simulink model "acf_sea_pad_research_20261006"  (R2026b)
settings: Solver=ode4  StopTime=p.stopTime  FixedStep=2.5000000000000002e-06
model workspace (MAT data in the model file):
  p : object (value not decoded)
  replayInputs = [0 0.0001 0.0002 0.0003 0.0004 0.0005 0.0006 0.0007 0.0008 0.0009 0.001 0.0011 ... (60003 elements, 20001x3)]
symbols that are objects in the model workspace (value not decoded): p
libraries: simulink x1
(part 2 of 2)

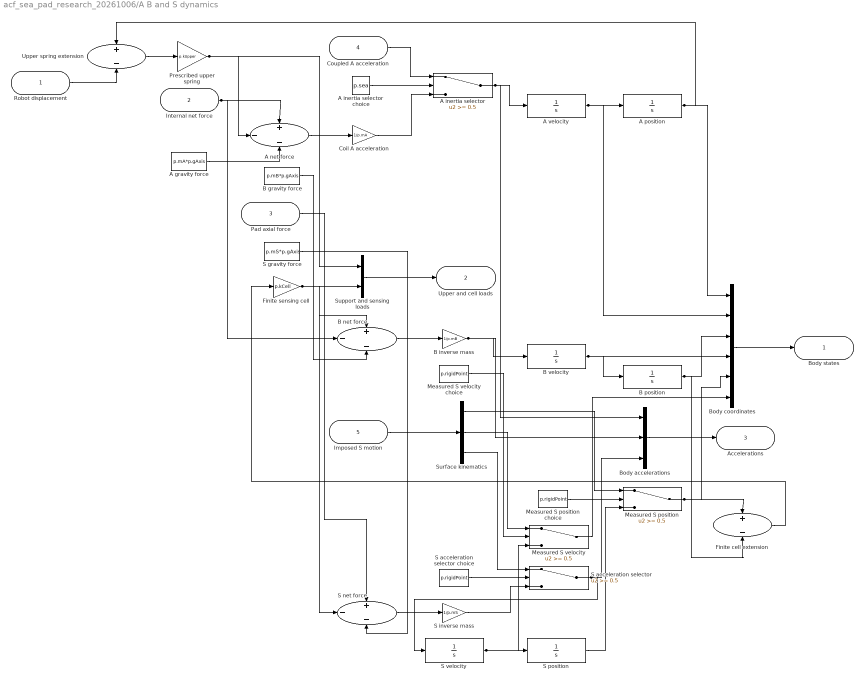
== system acf_sea_pad_research_20261006/A B and S dynamics ==
  Robot displacement : Inport
  Internal net force : Inport  Port=2
  Pad axial force : Inport  Port=3
  Coupled A acceleration : Inport  Port=4
  Imposed S motion : Inport  Port=5
  A gravity force : Constant  Value=p.mA*p.gAxis
  A inertia selector : Switch  Threshold=0.5  SaturateOnIntegerOverflow=off  InputSameDT=off
  A inertia selector choice : Constant  Value=p.sea
  A net force : Sum  Inputs=+--
  A position : Integrator  InitialCondition=p.initial(1)
  A velocity : Integrator  InitialCondition=p.initial(2)
  B gravity force : Constant  Value=p.mB*p.gAxis
  B inverse mass : Gain  Gain=1/p.mB
  B net force : Sum  Inputs=+--
  B position : Integrator  InitialCondition=p.initial(3)
  B velocity : Integrator  InitialCondition=p.initial(4)
  Body accelerations : Mux  Inputs=3
  Body coordinates : Mux  Inputs=6
  Coil A acceleration : Gain  Gain=1/p.mA
  Finite cell extension : Sum  Inputs=+-
  Finite sensing cell : Gain  Gain=p.kCell
  Measured S position : Switch  Threshold=0.5  SaturateOnIntegerOverflow=off  InputSameDT=off
  Measured S position choice : Constant  Value=p.rigidPoint
  Measured S velocity : Switch  Threshold=0.5  SaturateOnIntegerOverflow=off  InputSameDT=off
  Measured S velocity choice : Constant  Value=p.rigidPoint
  Prescribed upper spring : Gain  Gain=p.kUpper
  S acceleration selector : Switch  Threshold=0.5  SaturateOnIntegerOverflow=off  InputSameDT=off
  S acceleration selector choice : Constant  Value=p.rigidPoint
  S gravity force : Constant  Value=p.mS*p.gAxis
  S inverse mass : Gain  Gain=1/p.mS
  S net force : Sum  Inputs=+--
  S position : Integrator  InitialCondition=p.initial(5)
  S velocity : Integrator  InitialCondition=p.initial(6)
  Support and sensing loads : Mux  Inputs=2
  Surface kinematics : Demux  Outputs=3
  Upper spring extension : Sum  Inputs=+-
  Body states : Outport
  Upper and cell loads : Outport  Port=2
  Accelerations : Outport  Port=3
  wires:
  Finite cell extension/1 -> Finite sensing cell/1
  Body accelerations/1 -> Accelerations/1
  B position/1 -> Body coordinates/3, Finite cell extension/2
  A position/1 -> Body coordinates/1, Upper spring extension/1
  S position/1 -> Measured S position/3
  Coil A acceleration/1 -> A inertia selector/3
  Finite sensing cell/1 -> Support and sensing loads/2, S net force/2, B net force/1
  Measured S velocity/1 -> Body coordinates/6
  A net force/1 -> Coil A acceleration/1
  A inertia selector/1 -> A velocity/1, Body accelerations/1
  Measured S position/1 -> Body coordinates/5, Finite cell extension/1
  A inertia selector choice/1 -> A inertia selector/2
  A gravity force/1 -> A net force/3
  S acceleration selector choice/1 -> S acceleration selector/2
  Support and sensing loads/1 -> Upper and cell loads/1
  Imposed S motion/1 -> Surface kinematics/1
  Measured S velocity choice/1 -> Measured S velocity/2
  Pad axial force/1 -> S net force/1
  Surface kinematics/2 -> Measured S velocity/1
  Coupled A acceleration/1 -> A inertia selector/1
  Prescribed upper spring/1 -> A net force/2, Support and sensing loads/1
  S velocity/1 -> Measured S velocity/3, S position/1
  Upper spring extension/1 -> Prescribed upper spring/1
  Robot displacement/1 -> Upper spring extension/2
  Surface kinematics/3 -> S acceleration selector/1
  Body coordinates/1 -> Body states/1
  S gravity force/1 -> S net force/3
  B net force/1 -> B inverse mass/1
  S inverse mass/1 -> S acceleration selector/3
  S net force/1 -> S inverse mass/1
  Internal net force/1 -> B net force/2, A net force/1
  B inverse mass/1 -> B velocity/1, Body accelerations/2
  Surface kinematics/1 -> Measured S position/1
  B gravity force/1 -> B net force/3
  A velocity/1 -> A position/1, Body coordinates/2
  B velocity/1 -> B position/1, Body coordinates/4
  S acceleration selector/1 -> Body accelerations/3, S velocity/1
  Measured S position choice/1 -> Measured S position/2

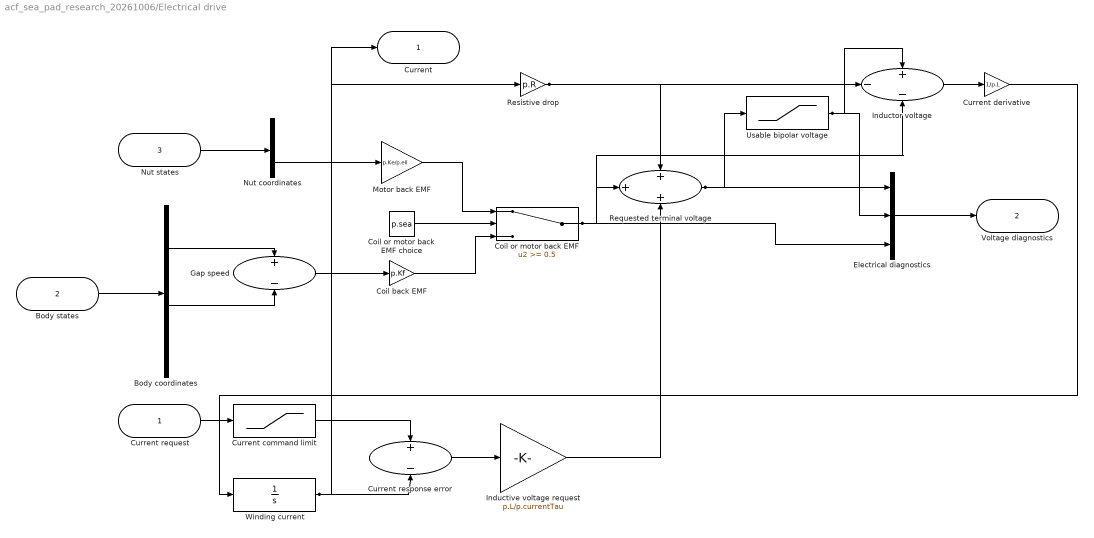
== system acf_sea_pad_research_20261006/Electrical drive ==
  Current request : Inport
  Body states : Inport  Port=2
  Nut states : Inport  Port=3
  Body coordinates : Demux  Outputs=6
  Coil back EMF : Gain  Gain=p.Kf
  Coil or motor back EMF : Switch  Threshold=0.5  SaturateOnIntegerOverflow=off  InputSameDT=off
  Coil or motor back EMF choice : Constant  Value=p.sea
  Current command limit : Saturate  UpperLimit=p.Imax  LowerLimit=-p.Imax
  Current derivative : Gain  Gain=1/p.L
  Current response error : Sum  Inputs=+-
  Electrical diagnostics : Mux  Inputs=3
  Gap speed : Sum  Inputs=+-
  Inductive voltage request : Gain  Gain=p.L/p.currentTau
  Inductor voltage : Sum  Inputs=+--
  Motor back EMF : Gain  Gain=p.Ke/p.ell
  Nut coordinates : Demux  Outputs=2
  Requested terminal voltage : Sum  Inputs=+++
  Resistive drop : Gain  Gain=p.R
  Usable bipolar voltage : Saturate  UpperLimit=p.Vmax  LowerLimit=-p.Vmax
  Winding current : Integrator  InitialCondition=p.initial(9)
  Current : Outport
  Voltage diagnostics : Outport  Port=2
  wires:
  Current derivative/1 -> Winding current/1
  Electrical diagnostics/1 -> Voltage diagnostics/1
  Inductor voltage/1 -> Current derivative/1
  Inductive voltage request/1 -> Requested terminal voltage/3
  Resistive drop/1 -> Requested terminal voltage/1, Inductor voltage/2
  Body states/1 -> Body coordinates/1
  Usable bipolar voltage/1 -> Electrical diagnostics/2, Inductor voltage/1
  Nut states/1 -> Nut coordinates/1
  Body coordinates/2 -> Gap speed/1
  Coil or motor back EMF/1 -> Requested terminal voltage/2, Inductor voltage/3, Electrical diagnostics/3
  Body coordinates/4 -> Gap speed/2
  Current request/1 -> Current command limit/1
  Current command limit/1 -> Current response error/1
  Nut coordinates/2 -> Motor back EMF/1
  Current response error/1 -> Inductive voltage request/1
  Gap speed/1 -> Coil back EMF/1
  Winding current/1 -> Current/1, Current response error/2, Resistive drop/1
  Coil or motor back EMF choice/1 -> Coil or motor back EMF/2
  Motor back EMF/1 -> Coil or motor back EMF/1
  Requested terminal voltage/1 -> Usable bipolar voltage/1, Electrical diagnostics/1
  Coil back EMF/1 -> Coil or motor back EMF/3

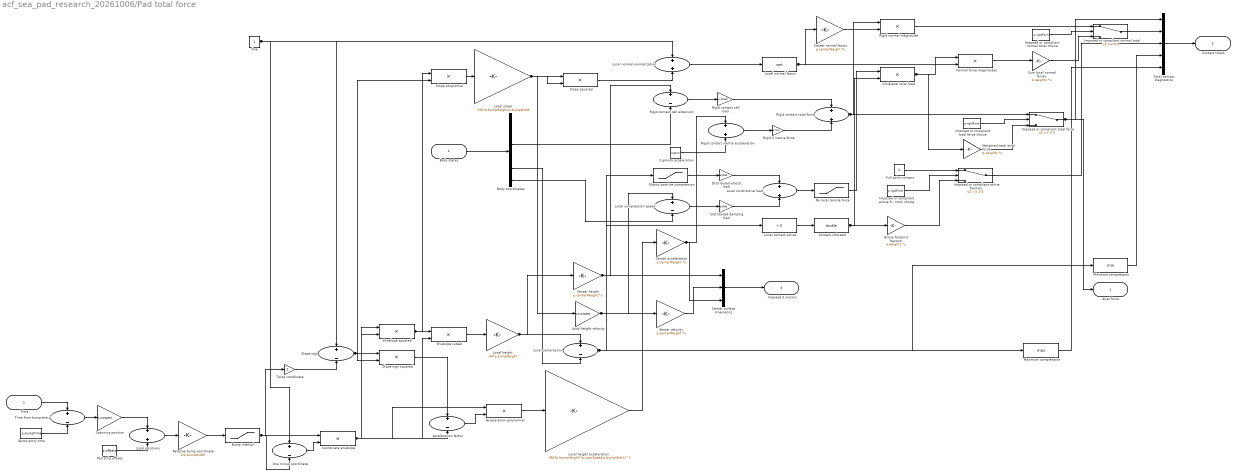
== system acf_sea_pad_research_20261006/Pad total force ==
  Time : Inport
  Body states : Inport  Port=2
  Acceleration factor : Sum  Inputs=+-
  Acceleration polynomial : Product  Inputs=**
  Active footprint fraction : Gain  Gain=p.weights  Multiplication=Matrix(K*u)
  Body coordinates : Demux  Outputs=6
  Bump entry time : Constant  Value=p.bumpTime
  Bump interval : Saturate  UpperLimit=1  LowerLimit=0
  Center acceleration : Gain  Gain=p.centerWeight  Multiplication=Matrix(K*u)
  Center height : Gain  Gain=p.centerWeight  Multiplication=Matrix(K*u)
  Center normal factor : Gain  Gain=p.centerWeight  Multiplication=Matrix(K*u)
  Center surface kinematics : Mux  Inputs=3
  Center velocity : Gain  Gain=p.centerWeight  Multiplication=Matrix(K*u)
  Contact indicator : DataTypeConversion  OutDataTypeStr=double  SaturateOnIntegerOverflow=off  RndMeth=Floor
  Coordinate envelope : Product  Inputs=**
  Distributed damping load : Gain  Gain=p.cPad
  Distributed elastic load : Gain  Gain=p.kPad
  Elastic positive compression : Saturate  UpperLimit=inf  LowerLimit=0
  Envelope cubed : Product  Inputs=**
  Envelope squared : Product  Inputs=**
  Full point contact : Constant
  Imposed or compliant active fraction : Switch  Threshold=0.5  SaturateOnIntegerOverflow=off  InputSameDT=off
  Imposed or compliant active fraction choice : Constant  Value=p.rigidPoint
  Imposed or compliant normal total : Switch  Threshold=0.5  SaturateOnIntegerOverflow=off  InputSameDT=off
  Imposed or compliant normal total choice : Constant  Value=p.rigidPoint
  Imposed or compliant total force : Switch  Threshold=0.5  SaturateOnIntegerOverflow=off  InputSameDT=off
  Imposed or compliant total force choice : Constant  Value=p.rigidPoint
  Local compression : Sum  Inputs=+-
  Local compression speed : Sum  Inputs=+-
  Local constitutive load : Sum
  Local contact active : simulink/Logic and Bit Operations/Compare To Constant  relop=>  const=0  OutDataTypeStr=boolean
  Local height : Gain  Gain=64*p.bumpHeight
  Local height acceleration : Gain  Gain=384*p.bumpHeight*(p.scanSpeed/p.bumpWidth)^2
  Local height velocity : Gain  Gain=p.scanSpeed
  Local normal factor : Sqrt
  Local normal normalization : Sum
  Local positions : Sum
  Local slope : Gain  Gain=192*p.bumpHeight/p.bumpWidth
  Maximum compression : MinMax  Function=max
  Minimum compression : MinMax
  No local tensile force : Saturate  UpperLimit=inf  LowerLimit=0
  Normal force magnitudes : Product  Inputs=**
  One : Constant
  One minus coordinate : Sum  Inputs=+-
  Pad strip offsets : Constant  Value=p.offsets
  Relative bump coordinate : Gain  Gain=1/p.bumpWidth
  Rigid S inertia force : Gain  Gain=p.mS
  Rigid contact cell extension : Sum  Inputs=+-
  Rigid contact cell load : Gain  Gain=p.kCell
  Rigid contact inertia acceleration : Sum
  Rigid contact total force : Sum
  Rigid normal magnitude : Product  Inputs=**
  S gravity acceleration : Constant  Value=p.gAxis
  Scanning position : Gain  Gain=p.scanSpeed
  Slope polynomial : Product  Inputs=**
  Slope sign : Sum  Inputs=+-
  Slope sign squared : Product  Inputs=**
  Slope squared : Product  Inputs=**
  Sum local normal forces : Gain  Gain=p.weights  Multiplication=Matrix(K*u)
  Time from bump entry : Sum  Inputs=+-
  Total contact diagnostics : Mux  Inputs=5
  Twice coordinate : Gain  Gain=2
  Unilateral local load : Product  Inputs=**
  Weighted total axial force : Gain  Gain=p.weights  Multiplication=Matrix(K*u)
  Axial force : Outport
  Contact totals : Outport  Port=2
  Imposed S motion : Outport  Port=3
  wires:
  Minimum compression/1 -> Total contact diagnostics/4
  Imposed or compliant normal total/1 -> Total contact diagnostics/2
  Maximum compression/1 -> Total contact diagnostics/5
  Local compression/1 -> Elastic positive compression/1, Maximum compression/1, Local contact active/1, Minimum compression/1
  Slope squared/1 -> Local normal normalization/2
  Acceleration polynomial/1 -> Local height acceleration/1
  Distributed damping load/1 -> Local constitutive load/2
  Local height/1 -> Center height/1, Local compression/1
  Elastic positive compression/1 -> Distributed elastic load/1
  Center acceleration/1 -> Center surface kinematics/3, Rigid contact inertia acceleration/1
  Center normal factor/1 -> Rigid normal magnitude/2
  Imposed or compliant active fraction choice/1 -> Imposed or compliant active fraction/2
  Slope polynomial/1 -> Local slope/1
  Local normal normalization/1 -> Local normal factor/1
  Envelope cubed/1 -> Local height/1
  Local contact active/1 -> Contact indicator/1
  Slope sign squared/1 -> Acceleration factor/1
  Normal force magnitudes/1 -> Sum local normal forces/1
  Imposed or compliant active fraction/1 -> Total contact diagnostics/3
  Sum local normal forces/1 -> Imposed or compliant normal total/3
  Time from bump entry/1 -> Scanning position/1
  Body coordinates/5 -> Local compression/2
  Body coordinates/3 -> Rigid contact cell extension/2
  Bump entry time/1 -> Time from bump entry/2
  Scanning position/1 -> Local positions/1
  Twice coordinate/1 -> Slope sign/2
  Total contact diagnostics/1 -> Contact totals/1
  Center height/1 -> Center surface kinematics/1, Rigid contact cell extension/1
  Pad strip offsets/1 -> Local positions/2
  Contact indicator/1 -> Active footprint fraction/1, Unilateral local load/2
  Local positions/1 -> Relative bump coordinate/1
  One minus coordinate/1 -> Coordinate envelope/2
  Relative bump coordinate/1 -> Bump interval/1
  Slope sign/1 -> Slope sign squared/2, Slope polynomial/2, Slope sign squared/1
  Local slope/1 -> Slope squared/2, Slope squared/1, Local height velocity/1
  Acceleration factor/1 -> Acceleration polynomial/2
  Bump interval/1 -> Twice coordinate/1, One minus coordinate/2, Coordinate envelope/1
  Time/1 -> Time from bump entry/1
  Imposed or compliant total force/1 -> Axial force/1, Total contact diagnostics/1
  Rigid contact inertia acceleration/1 -> Rigid S inertia force/1
  Coordinate envelope/1 -> Envelope squared/1, Acceleration factor/2, Envelope squared/2, Acceleration polynomial/1, Envelope cubed/2
  Envelope squared/1 -> Slope polynomial/1, Envelope cubed/1
  Body states/1 -> Body coordinates/1
  Local normal factor/1 -> Center normal factor/1, Normal force magnitudes/2
  Active footprint fraction/1 -> Imposed or compliant active fraction/3
  Local height acceleration/1 -> Center acceleration/1
  One/1 -> Slope sign/1, Local normal normalization/1, One minus coordinate/1
  Center surface kinematics/1 -> Imposed S motion/1
  S gravity acceleration/1 -> Rigid contact inertia acceleration/2
  Local constitutive load/1 -> No local tensile force/1
  Local compression speed/1 -> Distributed damping load/1
  Rigid S inertia force/1 -> Rigid contact total force/2
  Center velocity/1 -> Center surface kinematics/2
  Unilateral local load/1 -> Normal force magnitudes/1, Weighted total axial force/1
  Imposed or compliant normal total choice/1 -> Imposed or compliant normal total/2
  Body coordinates/6 -> Local compression speed/2
  Rigid contact cell load/1 -> Rigid contact total force/1
  Distributed elastic load/1 -> Local constitutive load/1
  Local height velocity/1 -> Center velocity/1, Local compression speed/1
  Rigid contact total force/1 -> Rigid normal magnitude/1, Imposed or compliant total force/1
  No local tensile force/1 -> Unilateral local load/1
  Weighted total axial force/1 -> Imposed or compliant total force/3
  Rigid normal magnitude/1 -> Imposed or compliant normal total/1
  Imposed or compliant total force choice/1 -> Imposed or compliant total force/2
  Rigid contact cell extension/1 -> Rigid contact cell load/1
  Full point contact/1 -> Imposed or compliant active fraction/1

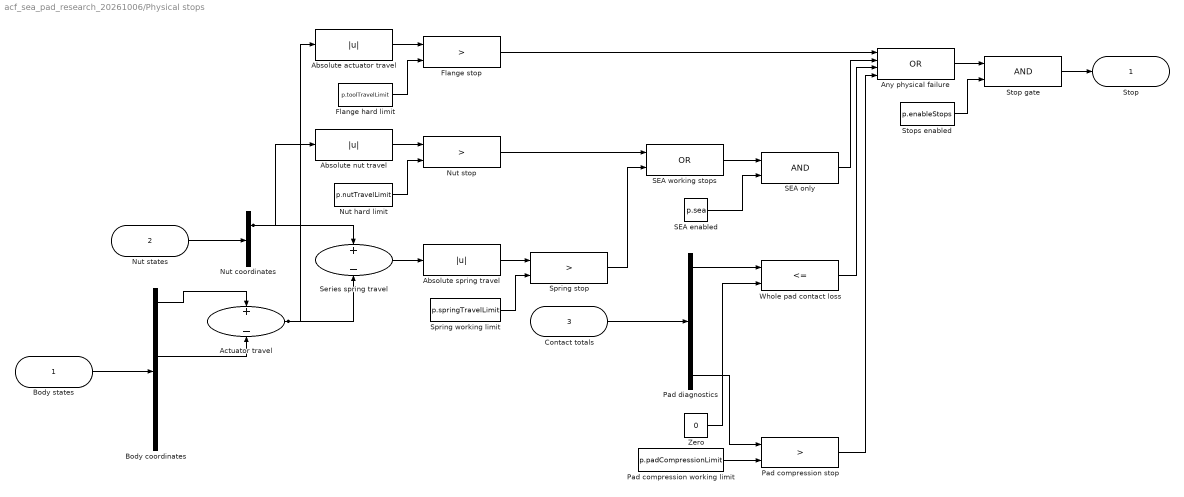
== system acf_sea_pad_research_20261006/Physical stops ==
  Body states : Inport
  Nut states : Inport  Port=2
  Contact totals : Inport  Port=3
  Absolute actuator travel : Abs  SaturateOnIntegerOverflow=off
  Absolute nut travel : Abs  SaturateOnIntegerOverflow=off
  Absolute spring travel : Abs  SaturateOnIntegerOverflow=off
  Actuator travel : Sum  Inputs=+-
  Any physical failure : Logic  Operator=OR  Inputs=4  AllPortsSameDT=off  OutDataTypeStr=boolean
  Body coordinates : Demux  Outputs=6
  Flange hard limit : Constant  Value=p.toolTravelLimit
  Flange stop : RelationalOperator  Operator=>  OutDataTypeStr=boolean  RndMeth=Simplest  InputSameDT=off
  Nut coordinates : Demux  Outputs=2
  Nut hard limit : Constant  Value=p.nutTravelLimit
  Nut stop : RelationalOperator  Operator=>  OutDataTypeStr=boolean  RndMeth=Simplest  InputSameDT=off
  Pad compression stop : RelationalOperator  Operator=>  OutDataTypeStr=boolean  RndMeth=Simplest  InputSameDT=off
  Pad compression working limit : Constant  Value=p.padCompressionLimit
  Pad diagnostics : Demux  Outputs=5
  SEA enabled : Constant  Value=p.sea
  SEA only : Logic  AllPortsSameDT=off  OutDataTypeStr=boolean
  SEA working stops : Logic  Operator=OR  AllPortsSameDT=off  OutDataTypeStr=boolean
  Series spring travel : Sum  Inputs=+-
  Spring stop : RelationalOperator  Operator=>  OutDataTypeStr=boolean  RndMeth=Simplest  InputSameDT=off
  Spring working limit : Constant  Value=p.springTravelLimit
  Stop gate : Logic  AllPortsSameDT=off  OutDataTypeStr=boolean
  Stops enabled : Constant  Value=p.enableStops
  Whole pad contact loss : RelationalOperator  Operator=<=  OutDataTypeStr=boolean  RndMeth=Simplest  InputSameDT=off
  Zero : Constant  Value=0
  Stop : Outport
  wires:
  Stop gate/1 -> Stop/1
  Pad compression stop/1 -> Any physical failure/4
  Whole pad contact loss/1 -> Any physical failure/3
  Any physical failure/1 -> Stop gate/1
  SEA only/1 -> Any physical failure/2
  Pad compression working limit/1 -> Pad compression stop/2
  Stops enabled/1 -> Stop gate/2
  SEA enabled/1 -> SEA only/2
  SEA working stops/1 -> SEA only/1
  Contact totals/1 -> Pad diagnostics/1
  Pad diagnostics/1 -> Whole pad contact loss/1
  Spring working limit/1 -> Spring stop/2
  Absolute spring travel/1 -> Spring stop/1
  Body states/1 -> Body coordinates/1
  Nut states/1 -> Nut coordinates/1
  Body coordinates/1 -> Actuator travel/1
  Body coordinates/3 -> Actuator travel/2
  Zero/1 -> Whole pad contact loss/2
  Nut stop/1 -> SEA working stops/1
  Pad diagnostics/5 -> Pad compression stop/1
  Actuator travel/1 -> Absolute actuator travel/1, Series spring travel/2
  Absolute actuator travel/1 -> Flange stop/1
  Flange hard limit/1 -> Flange stop/2
  Series spring travel/1 -> Absolute spring travel/1
  Nut coordinates/1 -> Absolute nut travel/1, Series spring travel/1
  Absolute nut travel/1 -> Nut stop/1
  Nut hard limit/1 -> Nut stop/2
  Spring stop/1 -> SEA working stops/2
  Flange stop/1 -> Any physical failure/1

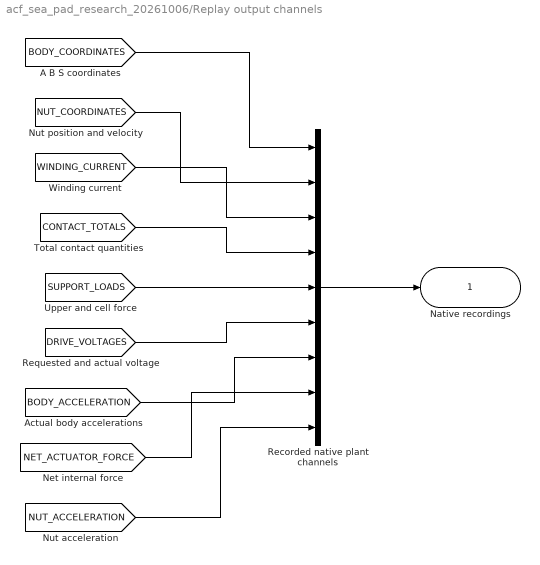
== system acf_sea_pad_research_20261006/Replay output channels ==
  Recorded native plant channels : Mux  Inputs=9
  Native recordings : Outport
  wires:
  Recorded native plant channels/1 -> Native recordings/1
  [NUT_ACCELERATION] -> Recorded native plant channels/9
  [NET_ACTUATOR_FORCE] -> Recorded native plant channels/8
  [DRIVE_VOLTAGES] -> Recorded native plant channels/6
  [SUPPORT_LOADS] -> Recorded native plant channels/5
  [CONTACT_TOTALS] -> Recorded native plant channels/4
  [BODY_ACCELERATION] -> Recorded native plant channels/7
  [WINDING_CURRENT] -> Recorded native plant channels/3
  [NUT_COORDINATES] -> Recorded native plant channels/2
  [BODY_COORDINATES] -> Recorded native plant channels/1

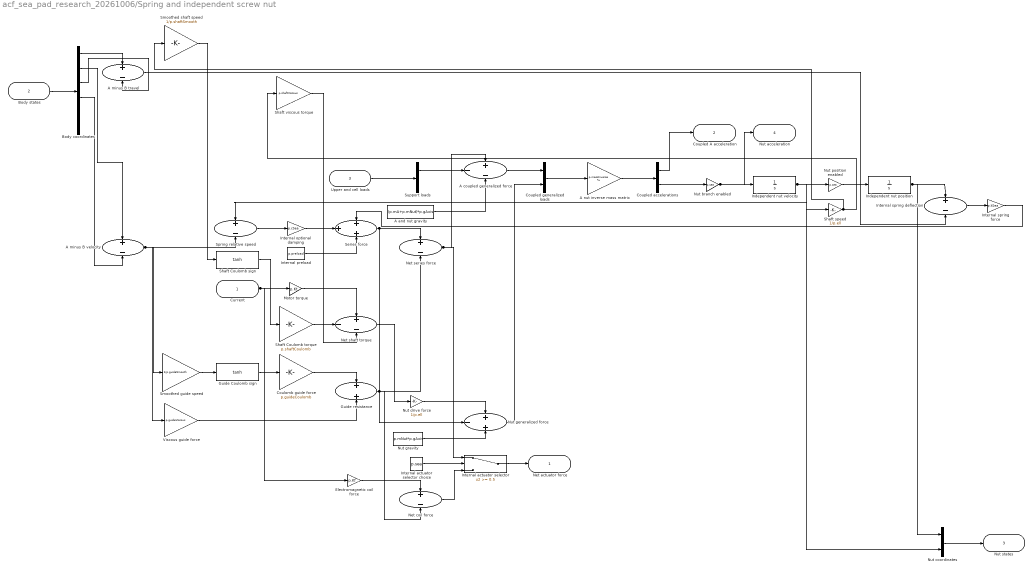
== system acf_sea_pad_research_20261006/Spring and independent screw nut ==
  Current : Inport
  Body states : Inport  Port=2
  Upper and cell loads : Inport  Port=3
  A and nut gravity : Constant  Value=(p.mA+p.mNut)*p.gAxis
  A coupled generalized force : Sum  Inputs=+--
  A minus B travel : Sum  Inputs=+-
  A minus B velocity : Sum  Inputs=+-
  A nut inverse mass matrix : Gain  Gain=p.massInverse  Multiplication=Matrix(K*u)
  Body coordinates : Demux  Outputs=6
  Coulomb guide force : Gain  Gain=p.guideCoulomb
  Coupled accelerations : Demux  Outputs=2
  Coupled generalized loads : Mux  Inputs=2
  Electromagnetic coil force : Gain  Gain=p.Kf
  Guide Coulomb sign : Trigonometry  Operator=tanh
  Guide resistance : Sum
  Independent nut position : Integrator  InitialCondition=p.initial(7)
  Independent nut velocity : Integrator  InitialCondition=p.initial(8)
  Internal actuator selector : Switch  Threshold=0.5  SaturateOnIntegerOverflow=off  InputSameDT=off
  Internal actuator selector choice : Constant  Value=p.sea
  Internal optional damping : Gain  Gain=p.cSea
  Internal preload : Constant  Value=p.preload
  Internal spring deflection : Sum  Inputs=+-
  Internal spring force : Gain  Gain=p.kSea
  Motor torque : Gain  Gain=p.Kt
  Net coil force : Sum  Inputs=+-
  Net series force : Sum  Inputs=+-
  Net shaft torque : Sum  Inputs=+--
  Nut branch enabled : Gain  Gain=p.sea
  Nut coordinates : Mux  Inputs=2
  Nut drive force : Gain  Gain=1/p.ell
  Nut generalized force : Sum  Inputs=+-+
  Nut gravity : Constant  Value=p.mNut*p.gAxis
  Nut position enabled : Gain  Gain=p.sea
  Series force : Sum  Inputs=+++
  Shaft Coulomb sign : Trigonometry  Operator=tanh
  Shaft Coulomb torque : Gain  Gain=p.shaftCoulomb
  Shaft speed : Gain  Gain=1/p.ell
  Shaft viscous torque : Gain  Gain=p.shaftViscous
  Smoothed guide speed : Gain  Gain=1/p.guideSmooth
  Smoothed shaft speed : Gain  Gain=1/p.shaftSmooth
  Spring relative speed : Sum  Inputs=+-
  Support loads : Demux  Outputs=2
  Viscous guide force : Gain  Gain=p.guideViscous
  Net actuator force : Outport
  Coupled A acceleration : Outport  Port=2
  Nut states : Outport  Port=3
  Nut acceleration : Outport  Port=4
  wires:
  Nut coordinates/1 -> Nut states/1
  Independent nut position/1 -> Nut coordinates/1, Internal spring deflection/1
  Nut position enabled/1 -> Independent nut position/1
  Independent nut velocity/1 -> Nut position enabled/1, Spring relative speed/1, Shaft speed/1, Nut coordinates/2
  Coupled accelerations/2 -> Nut branch enabled/1
  Coupled accelerations/1 -> Coupled A acceleration/1
  Shaft speed/1 -> Shaft viscous torque/1, Smoothed shaft speed/1
  A nut inverse mass matrix/1 -> Coupled accelerations/1
  Internal actuator selector/1 -> Net actuator force/1
  Nut generalized force/1 -> Coupled generalized loads/2
  A coupled generalized force/1 -> Coupled generalized loads/1
  Internal spring force/1 -> Series force/1
  Net coil force/1 -> Internal actuator selector/3
  Coupled generalized loads/1 -> A nut inverse mass matrix/1
  Nut gravity/1 -> Nut generalized force/3
  Current/1 -> Motor torque/1, Electromagnetic coil force/1
  Smoothed guide speed/1 -> Guide Coulomb sign/1
  Body coordinates/4 -> A minus B velocity/2
  Internal spring deflection/1 -> Internal spring force/1
  Motor torque/1 -> Net shaft torque/1
  Guide resistance/1 -> Net series force/2, Net coil force/2
  Viscous guide force/1 -> Guide resistance/2
  Net series force/1 -> Internal actuator selector/1, A coupled generalized force/1
  A minus B velocity/1 -> Viscous guide force/1, Smoothed guide speed/1, Spring relative speed/2
  Body coordinates/2 -> A minus B velocity/1
  Upper and cell loads/1 -> Support loads/1
  Nut drive force/1 -> Nut generalized force/1
  Body coordinates/3 -> A minus B travel/2
  Body coordinates/1 -> A minus B travel/1
  A minus B travel/1 -> Internal spring deflection/2
  Body states/1 -> Body coordinates/1
  Shaft Coulomb sign/1 -> Shaft Coulomb torque/1
  Shaft viscous torque/1 -> Net shaft torque/3
  Spring relative speed/1 -> Internal optional damping/1
  Internal preload/1 -> Series force/3
  Nut branch enabled/1 -> Nut acceleration/1, Independent nut velocity/1
  Shaft Coulomb torque/1 -> Net shaft torque/2
  Internal optional damping/1 -> Series force/2
  Series force/1 -> Net series force/1, Nut generalized force/2
  Internal actuator selector choice/1 -> Internal actuator selector/2
  A and nut gravity/1 -> A coupled generalized force/3
  Coulomb guide force/1 -> Guide resistance/1
  Smoothed shaft speed/1 -> Shaft Coulomb sign/1
  Electromagnetic coil force/1 -> Net coil force/1
  Guide Coulomb sign/1 -> Coulomb guide force/1
  Net shaft torque/1 -> Nut drive force/1
  Support loads/1 -> A coupled generalized force/2
